simulink model "PVonGrid_patched"  (R2025a)
settings: Solver=VariableStepAuto  StartTime=0.0  StopTime=2.0  RelTol=1e-3
PreLoadFcn:
  | % Parameter basis-watt yang menghasilkan Gambar 6 pada naskah.
  | % Sama persis dengan matlab/siapkan_workspace.m. JANGAN pakai
  | % init_VIC.m: nilainya set per-unit lama dan menghasilkan respons
  | % yang sama sekali berbeda.
  | f0 = 50;  Kw = 1;  H = 4;  Ts = 1e-5;
  | num_Tdi = 1;     den_Tdi    = [0.01 1];
  | num_Tri = 1;     den_Tri    = [0.01 1];
  | num_filter = 1;  den_filter = [0.02 1];
  | Dv = 20000;      Kiv = 632;
  | clear Prated R T_filter Tdi Tri VIC_max VIC_min
undefined symbols (not defined in the file): DiscIntNeverNeededParam, Down, Ion, Lithium, Up
libraries: spsSeriesRLCBranchLib x15, mcbeeMathTransformLib x8, spsIGBTDiodeLib x5, spsCurrentMeasurementLib x4, spsVoltageMeasurementLib x4, slpidlib x3, spsThreePhaseVIMeasurementLib x3, spsMosfetLib x2, spsDiodeLib x2, spsGroundLib x2, spsUniversalBridgeLib x2, spsPower3phInstantaneousLib x2
(part 1 of 2)
settings Model: Creator=Aryo  LastModifiedBy=ASUS

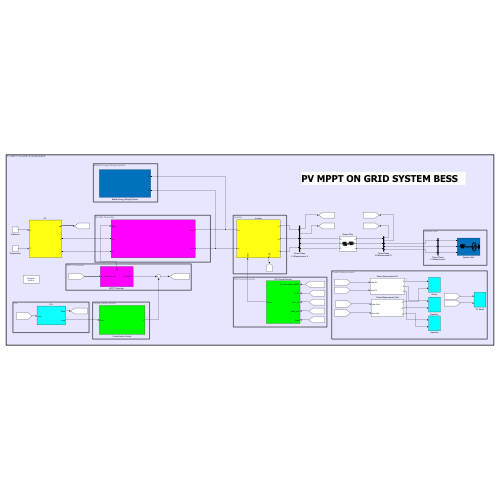
[thumbnail: Simulink's stored preview of the top-level diagram]
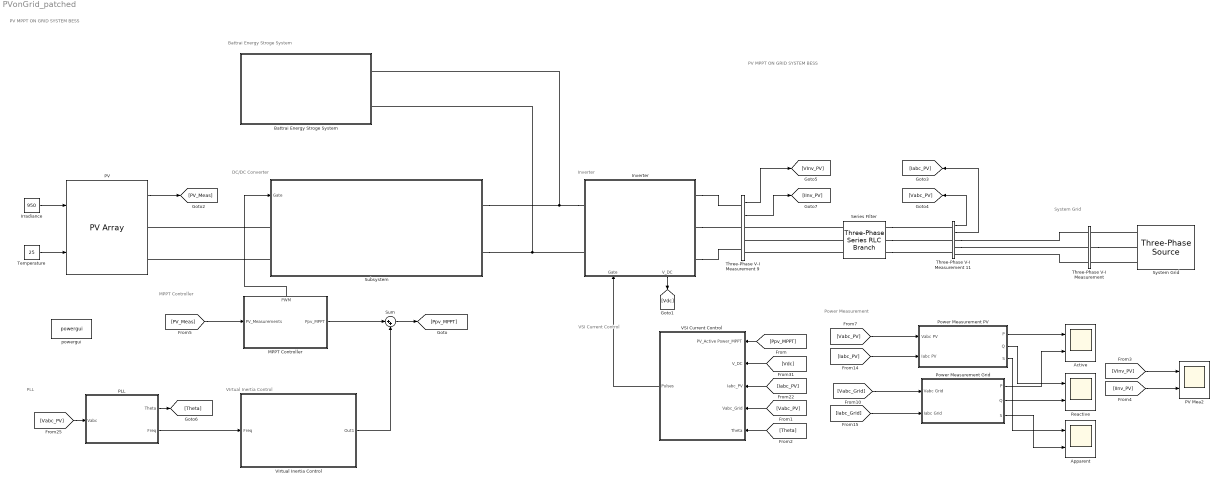
== system PVonGrid_patched ==
  note: PV MPPT ON GRID SYSTEM BESS
  note: PV MPPT ON GRID SYSTEM BESS
  note: VSI Current Control
  note: PLL
  note: Inverter
  note: Power Measurement
  note: MPPT Controller
  note: DC/DC Converter
  note: VIrtual Inertia Control
  note: Battrai Energy Stroge System
  note: System Grid
  "Active " : Scope  NumInputPorts=2
      settings: ActiveDisplayYMinimum=-60306.25275  ActiveDisplayYMaximum=6695.82422  DataLoggingVariableName=ScopeData8
  Apparent : Scope  NumInputPorts=2
      settings: ActiveDisplayYMinimum=-6789.47164  ActiveDisplayYMaximum=61149.07953  DataLoggingVariableName=ScopeData2
  Battrai Energy Stroge System : Subsystem
  Inverter : Subsystem
      settings: PortSchema="{\"entries\":[{\"content\":{\"sides\":[{\"content\":{\"connectorIds\":[\"LConn1\",\"LConn2\"]},\"type\":\"ConnectorPlacement.EquallySpacedRectSide\",\"uuid\":\"8d032cf4-7652-4960-826c-254f99f7bea5\"},{\"content\":{\"connectorIds\":[\"RConn1\",\"RConn2\",\"RConn3\"],\"side\":\"RIGHT\"},\"type\":\"ConnectorPlacement.EquallySpacedRectSide\",\"uuid\":\"6237d52f-d9ad-4fa0-b895-4b87ccfefd8d\"},{\"content\":{\"side\":\"TOP\"},\"type\":\"ConnectorPlacement.EquallySpacedRectSide\",\"uuid\":\"9697b938-6aa4-467c-bc3c-4144909828be\"},{\"content\":{\"connectorIds\":[\"In1\",\"Out1\"],\"side\":\"BOTTOM\"},\"type\":\"ConnectorPlacement.EquallySpacedRectSide\",\"uuid\":\"151792d3-0b7b-426c-bbcc-91f0e747f4d6\"}]},\"type\":\"ConnectorPlacement.EquallySpacedConnector\",\"uuid\":\"8854265a-e38a-4272-8fdc-bb8cf1e7f552\"}],\"packageUris\":[\"http://schema.mathworks.com/mf0/Connector/R2020b\"],\"version\":\"1.0\"}"
  "Irradiance " : Constant  Value=950
  MPPT Controller : Subsystem
      settings: PortSchema="{\"entries\":[{\"content\":{\"sides\":[{\"content\":{\"connectorIds\":[\"In1\"]},\"type\":\"ConnectorPlacement.EquallySpacedRectSide\",\"uuid\":\"beb56f4d-244a-4861-aa2c-056548243ef9\"},{\"content\":{\"connectorIds\":[\"Out1\"],\"side\":\"RIGHT\"},\"type\":\"ConnectorPlacement.EquallySpacedRectSide\",\"uuid\":\"efb26265-76c3-4ef7-8964-6d49d0ce5848\"},{\"content\":{\"connectorIds\":[\"Out2\"],\"side\":\"TOP\"},\"type\":\"ConnectorPlacement.EquallySpacedRectSide\",\"uuid\":\"f52004c3-ad48-43ff-bda9-03bf57742bdf\"}]},\"type\":\"ConnectorPlacement.EquallySpacedConnector\",\"uuid\":\"0b23e1d0-3529-41b8-bd5c-87ef798e8ebf\"}],\"packageUris\":[\"http://schema.mathworks.com/mf0/Connector/R2020b\"],\"version\":\"1.0\"}"
  PLL : Subsystem
  "PV " : spsPVArrayLib/PV Array  Npar=18  Nser=20  PlotType=array @ 1000 W/m2 & specified temperatures  S_vec="[ 1000  500  100 ]"  Temp_C_vec=[ 0 15 25 35 50]  ModuleName=User-defined  PlotWhenSelected=off  Pm=349.972  Ncell=96  Voc=51.7  Isc=8.65  Vm=43.1  Im=8.12  beta_Voc_pc=-0.37  alpha_Isc_pc=0.07  beta_Voc=-0.19129  alpha_Isc=0.006055  IL=8.6554  I0=4.1764e-10  nI=0.88295  Rsh=412.0293  Rs=0.25518  RobustModel=off  RobustCellTemperature=313.3991  BAL=on  Tc=1e-6  Tfilter=5e-5
  PV Mea2 : Scope  NumInputPorts=2
      settings: ActiveDisplayYMinimum=-434.46354  ActiveDisplayYMaximum=444.89351  DataLoggingVariableName=ScopeData15
  Power Measurement Grid : Subsystem
  Power Measurement PV : Subsystem
  "Reactive " : Scope  NumInputPorts=2
      settings: ActiveDisplayYMinimum=-15111.35327  ActiveDisplayYMaximum=19095.7131
  Series FIlter : spsThreePhaseSeriesRLCBranchLib/Three-Phase Series RLC Branch  LConnTagsString=A|B|C  RConnTagsString=A|B|C  BranchType=RL  Resistance=2.119394542  Inductance=10.59697271e-3  Capacitance=1e-6  Measurements=None
  Subsystem : Subsystem
  Sum : Sum  Inputs=|++
  System Grid : spsThreePhaseSourceLib/Three-Phase Source  InternalConnection=Yg  VoltagePhases=on  Voltage=380  PhaseAngle=0  Voltage_phases=[380 380 380]/sqrt(3)  PhaseAngles_phases=[0 -120 +120]  Frequency=50  NonIdealSource=on  SpecifyImpedance=off  Resistance=0  Inductance=6.56e-3  ShortCircuitLevel=100e6  BaseVoltage=380  XRratio=7  BusType=swing  Pref=1e6  Qref=0  Prefabc=[10e3, 10e3, 10e3]  Qrefabc=[0, 0, 0]  Qmin=-inf  Qmax=inf
  "Temperature " : Constant  Value=25
  "Three-Phase V-I Measurement " : spsThreePhaseVIMeasurementLib/Three-Phase V-I Measurement  VoltageMeasurement=phase-to-ground  SetLabelV=on  LabelV=Vabc_Grid  Vpu=off  VpuLL=off  CurrentMeasurement=yes  SetLabelI=on  LabelI=Iabc_Grid  Ipu=off  Pbase=100e6  Vbase=500e3  OutputType=Complex  PhasorSimulation=off  PSBequivalent=0
  Three-Phase V-I Measurement 11 : spsThreePhaseVIMeasurementLib/Three-Phase V-I Measurement  VoltageMeasurement=phase-to-ground  SetLabelV=off  LabelV=Vabc_PV  Vpu=off  VpuLL=off  CurrentMeasurement=yes  SetLabelI=off  LabelI=Iabc_PV  Ipu=off  Pbase=100e6  Vbase=500e3  OutputType=Complex  PhasorSimulation=off  PSBequivalent=0
  Three-Phase V-I Measurement 9 : spsThreePhaseVIMeasurementLib/Three-Phase V-I Measurement  VoltageMeasurement=phase-to-ground  SetLabelV=off  LabelV=VInv_PV  Vpu=off  VpuLL=off  CurrentMeasurement=yes  SetLabelI=off  LabelI=IInv_PV  Ipu=off  Pbase=100e6  Vbase=500e3  OutputType=Complex  PhasorSimulation=off  PSBequivalent=0
  VIrtual Inertia Control : Subsystem
  "VSI Current Control " : Subsystem
  powergui : sps_lib/powergui  Priority=1  SimulationMode=Discrete  SampleTime=1e-6  frequency=60  Iterations=50  frequencyindice=50  Pbase=100e6  ErrMax=1e-4  UnitsV=kV  UnitsW=MW  buscounter=0  FunctionMessages=off  echomessages=off  EnableUseOfTLC=off  CurrentSourceSwitches=off  DisableSnubberDevices=off  DisableRonSwitches=off  DisableVfSwitches=off  DisplayEquations=off  AutomaticDiscreteSolvers=off  SolverType=Tustin/Backward Euler (TBE)  Interpol=off  ExternalGateDelay=off  methode=off  Ts=100  x0status=blocks  SPID=on  SwTol=0  HookPort=off  NonlinearTolerance=1e-4  nMaxIteration=100  ContinueOnMaxIteration=off  RestoreLinks=warning  ResistiveCurrentMeasurement=off  Frange=[0:2:500]  Ylog=off  Xlog=on  ShowGrid=off  save=off  variable=ZData  structure=0  ZoomFFT=off  StartTime=0.0  cycles=1  DisplayStyle=1  fundamental=60  FreqAxis=off  MaxFrequency=1000  frequencyindicesteady=1  RmsSteady=1  display=off
  wires:
  Power Measurement Grid/1(P) -> "Active "/2
  Power Measurement Grid/3(S) -> Apparent/2
  Power Measurement Grid/2(Q) -> "Reactive "/2
  [Vabc_PV] -> Power Measurement PV/1(Vabc PV)
  [Vabc_PV] -> PLL/1(Vabc)
  [Theta] -> "VSI Current Control "/5(Theta)
  [Iabc_PV] -> "VSI Current Control "/3(Iabc_PV)
  [Iabc_PV] -> Power Measurement PV/2(Iabc PV)
  [Ppv_MPPT] -> "VSI Current Control "/1(PV_Active Power_MPPT)
  Sum/1 -> [Ppv_MPPT]
  [Vdc] -> "VSI Current Control "/2(V_DC)
  [Vabc_PV] -> "VSI Current Control "/4(Vabc_Grid)
  MPPT Controller/1(Ppv_MPPT) -> Sum/1
  VIrtual Inertia Control/1(Out1) -> Sum/2
  PLL/1(Theta) -> [Theta]
  Three-Phase V-I Measurement 11/1 -> [Vabc_PV]
  [Vabc_Grid] -> Power Measurement Grid/1(Vabc Grid)
  Inverter/1(V_DC) -> [Vdc]
  Three-Phase V-I Measurement 11/2 -> [Iabc_PV]
  Three-Phase V-I Measurement 9/2 -> [IInv_PV]
  "Irradiance "/1 -> "PV "/1
  PLL/2(Freq) -> VIrtual Inertia Control/1(Freq)
  [Iabc_Grid] -> Power Measurement Grid/2(Iabc Grid)
  "PV "/1 -> [PV_Meas]
  Three-Phase V-I Measurement 9/1 -> [VInv_PV]
  "Temperature "/1 -> "PV "/2
  Power Measurement PV/2(Q) -> "Reactive "/1
  Power Measurement PV/3(S) -> Apparent/1
  "VSI Current Control "/1(Pulses) -> Inverter/1(Gate)
  [PV_Meas] -> MPPT Controller/1(PV_Measurements)
  Power Measurement PV/1(P) -> "Active "/1
  [VInv_PV] -> PV Mea2/1
  [IInv_PV] -> PV Mea2/2
  MPPT Controller/2(PWM) -> Subsystem/1(Gate)
  connections:
  Subsystem/RConn2 -- Battrai Energy Stroge System/RConn2 -- Inverter/LConn2
  Inverter/LConn1 -- Subsystem/RConn1 -- Battrai Energy Stroge System/RConn1
  Series FIlter/RConn2 -- Three-Phase V-I Measurement 11/LConn2
  Inverter/RConn2 -- Three-Phase V-I Measurement 9/LConn2
  Inverter/RConn1 -- Three-Phase V-I Measurement 9/LConn1
  Series FIlter/RConn3 -- Three-Phase V-I Measurement 11/LConn3
  Series FIlter/LConn1 -- Three-Phase V-I Measurement 9/RConn1
  Series FIlter/LConn2 -- Three-Phase V-I Measurement 9/RConn2
  Series FIlter/LConn3 -- Three-Phase V-I Measurement 9/RConn3
  "Three-Phase V-I Measurement "/LConn3 -- Three-Phase V-I Measurement 11/RConn3
  Inverter/RConn3 -- Three-Phase V-I Measurement 9/LConn3
  Three-Phase V-I Measurement 11/RConn1 -- "Three-Phase V-I Measurement "/LConn1
  Three-Phase V-I Measurement 11/RConn2 -- "Three-Phase V-I Measurement "/LConn2
  System Grid/RConn3 -- "Three-Phase V-I Measurement "/RConn3
  Series FIlter/RConn1 -- Three-Phase V-I Measurement 11/LConn1
  "Three-Phase V-I Measurement "/RConn2 -- System Grid/RConn2
  System Grid/RConn1 -- "Three-Phase V-I Measurement "/RConn1
  Subsystem/LConn1 -- "PV "/RConn1
  Subsystem/LConn2 -- "PV "/RConn2

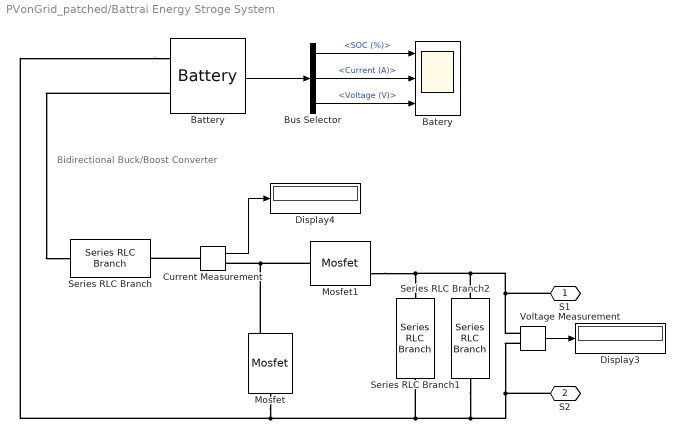
== system PVonGrid_patched/Battrai Energy Stroge System ==
  note: Bidirectional Buck/Boost Converter
  Batery : Scope  NumInputPorts=3
      settings: ActiveDisplayYMinimum=99.98642  ActiveDisplayYMaximum=100.00151  DataLoggingVariableName=ScopeData12
  Battery : spsBatteryLib/Battery  BatType=Lithium-Ion  NomV=400  NomQ=150  SOC=100  Batt_Tr=30  PresetModel=on  MaxQ=150  MinV=300  FullV=465.5949  Dis_rate=65.2174  R=0.026667  Normal_OP=135.6522  expZone="[432.1543      7.369565]"
  Bus Selector : BusSelector  OutputSignals=SOC (%),Current (A),Voltage (V)
  Current Measurement : spsCurrentMeasurementLib/Current Measurement  PhasorSimulation=off  OutputType=Complex  PSBequivalent=0
  Display3 : Display
  Display4 : Display
  Mosfet : spsMosfetLib/Mosfet  Ron=0.1  Lon=0  Rd=0.01  Vfd=0  IC=0  Rs=1e5  Cs=inf  Measurements=off
  Mosfet1 : spsMosfetLib/Mosfet  Ron=0.1  Lon=0  Rd=0.01  Vfd=0  IC=0  Rs=1e5  Cs=inf  Measurements=off
  Series RLC Branch : spsSeriesRLCBranchLib/Series RLC Branch  LConnTagsString=__new0  RConnTagsString=__new0  BranchType=L  Resistance=1  Inductance=1e-3  SetiL0=off  InitialCurrent=0  Capacitance=1e-6  Setx0=off  InitialVoltage=0  Measurements=None
  Series RLC Branch1 : spsSeriesRLCBranchLib/Series RLC Branch  LConnTagsString=__new0  RConnTagsString=__new0  BranchType=RC  Resistance=1  Inductance=1e-3  SetiL0=off  InitialCurrent=0  Capacitance=1e-6  Setx0=off  InitialVoltage=0  Measurements=None
  Series RLC Branch2 : spsSeriesRLCBranchLib/Series RLC Branch  LConnTagsString=__new0  RConnTagsString=__new0  BranchType=R  Resistance=1  Inductance=1e-3  SetiL0=off  InitialCurrent=0  Capacitance=1e-6  Setx0=off  InitialVoltage=0  Measurements=None
  Voltage Measurement : spsVoltageMeasurementLib/Voltage Measurement  PhasorSimulation=off  OutputType=Complex  PSBequivalent=0
  S1 : PMIOPort  Side=Right
  S2 : PMIOPort  Port=2  Side=Right
  wires:
  Battery/1 -> Bus Selector/1
  Voltage Measurement/1 -> Display3/1
  Current Measurement/1 -> Display4/1
  Bus Selector/3 -> Batery/3  "<Voltage (V)>"
  Bus Selector/1 -> Batery/1  "<SOC (%)>"
  Bus Selector/2 -> Batery/2  "<Current (A)>"
  connections:
  Current Measurement/RConn1 -- Mosfet/LConn1 -- Mosfet1/RConn1
  Battery/LConn2 -- Mosfet/RConn1 -- Series RLC Branch1/RConn1 -- Voltage Measurement/LConn2 -- S2/RConn1 -- Series RLC Branch2/RConn1
  S1/RConn1 -- Series RLC Branch2/LConn1 -- Series RLC Branch1/LConn1 -- Mosfet1/LConn1 -- Voltage Measurement/LConn1
  Battery/LConn1 -- Series RLC Branch/LConn1
  Current Measurement/LConn1 -- Series RLC Branch/RConn1

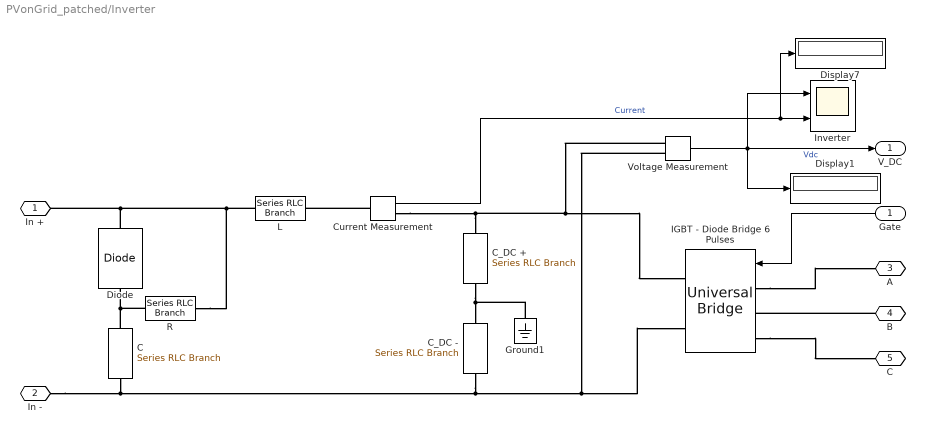
== system PVonGrid_patched/Inverter ==
  Gate : Inport
  "C " : spsSeriesRLCBranchLib/Series RLC Branch  LConnTagsString=__new0  RConnTagsString=__new0  BranchType=RC  Resistance=3e-3  Inductance=1e-3  SetiL0=off  InitialCurrent=0  Capacitance=200e-6  Setx0=off  InitialVoltage=0  Measurements=None
  C_DC + : spsSeriesRLCBranchLib/Series RLC Branch  LConnTagsString=__new0  RConnTagsString=__new0  BranchType=RC  Resistance=1e-3  Inductance=1e-3  SetiL0=off  InitialCurrent=0  Capacitance=1500e-6  Setx0=off  InitialVoltage=0  Measurements=None
  C_DC - : spsSeriesRLCBranchLib/Series RLC Branch  LConnTagsString=__new0  RConnTagsString=__new0  BranchType=RC  Resistance=1e-3  Inductance=1e-3  SetiL0=off  InitialCurrent=0  Capacitance=1500e-6  Setx0=off  InitialVoltage=0  Measurements=None
  "Current Measurement " : spsCurrentMeasurementLib/Current Measurement  PhasorSimulation=off  OutputType=Complex  PSBequivalent=0
  "Diode " : spsDiodeLib/Diode  Ron=0.001  Lon=0  Vf=1.5  IC=0  UseSnubber=0  Rs=500  Cs=250e-9  Measurements=off
  Display1 : Display
  Display7 : Display
  Ground1 : spsGroundLib/Ground  LConnTagsString=a
  IGBT - Diode Bridge 6 Pulses : spsUniversalBridgeLib/Universal Bridge  Arms=3  SnubberResistance=1e5  SnubberCapacitance=inf  Device=IGBT / Diodes  Ron=2.5e-3  Lon=0  ForwardVoltages="[  2.2  1.5  ]"  ForwardVoltage=0  GTOparameters=[ 10e-6 , 20e-6 ]  IGBTparameters=[ 1e-6 , 2e-6 ]  Measurements=None  Measurements_2=None  converterType=Rectifier
  Inverter : Scope  NumInputPorts=2
      settings: ActiveDisplayYMinimum=-86.61598  ActiveDisplayYMaximum=779.54311  DataLoggingVariableName=ScopeData11
  L : spsSeriesRLCBranchLib/Series RLC Branch  LConnTagsString=__new0  RConnTagsString=__new0  BranchType=RL  Resistance=5  Inductance=25e-3  SetiL0=off  InitialCurrent=0  Capacitance=5000e-6  Setx0=off  InitialVoltage=0  Measurements=None
  R : spsSeriesRLCBranchLib/Series RLC Branch  LConnTagsString=__new0  RConnTagsString=__new0  BranchType=R  Resistance=2  Inductance=5e-3  SetiL0=off  InitialCurrent=0  Capacitance=5000e-6  Setx0=off  InitialVoltage=0  Measurements=None
  "Voltage Measurement " : spsVoltageMeasurementLib/Voltage Measurement  PhasorSimulation=off  OutputType=Complex  PSBequivalent=0
  In + : PMIOPort  Side=Left
  In - : PMIOPort  Port=2  Side=Left
  A : PMIOPort  Port=3  Side=Right
  B : PMIOPort  Port=4  Side=Right
  C : PMIOPort  Port=5  Side=Right
  V_DC : Outport
  wires:
  Gate/1 -> IGBT - Diode Bridge 6 Pulses/1
  "Current Measurement "/1 -> Display7/1, Inverter/2  "Current"
  "Voltage Measurement "/1 -> Display1/1, Inverter/1, V_DC/1  "Vdc"
  connections:
  C_DC +/RConn1 -- Ground1/LConn1 -- C_DC -/LConn1
  L/LConn1 -- R/RConn1 -- "Diode "/LConn1 -- In +/RConn1
  C_DC +/LConn1 -- "Current Measurement "/RConn1 -- IGBT - Diode Bridge 6 Pulses/RConn1 -- "Voltage Measurement "/LConn1
  IGBT - Diode Bridge 6 Pulses/LConn1 -- A/RConn1
  IGBT - Diode Bridge 6 Pulses/LConn3 -- C/RConn1
  In -/RConn1 -- "C "/RConn1 -- C_DC -/RConn1 -- IGBT - Diode Bridge 6 Pulses/RConn2 -- "Voltage Measurement "/LConn2
  B/RConn1 -- IGBT - Diode Bridge 6 Pulses/LConn2
  "Current Measurement "/LConn1 -- L/RConn1
  "Diode "/RConn1 -- "C "/LConn1 -- R/LConn1

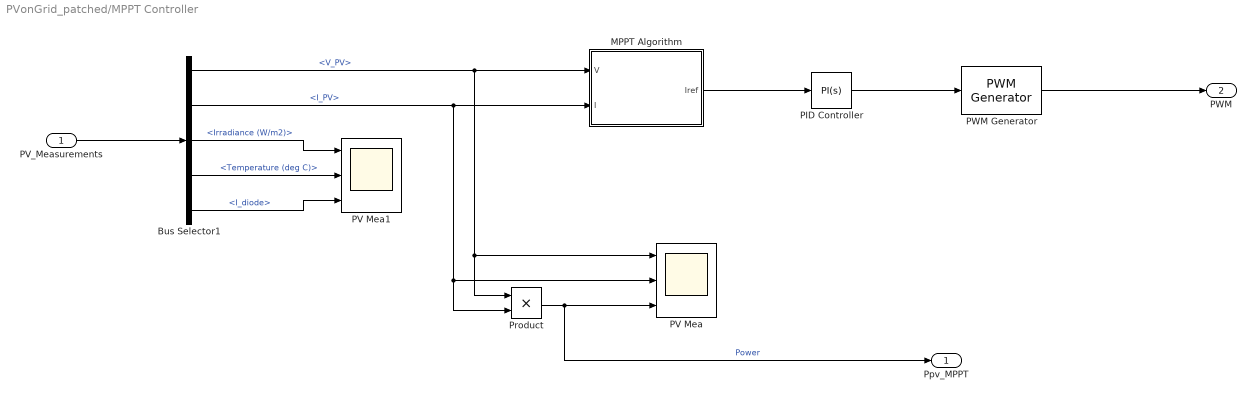
== system PVonGrid_patched/MPPT Controller ==
  PV_Measurements : Inport
  Bus Selector1 : BusSelector  OutputSignals=V_PV,I_PV,Irradiance (W/m2),Temperature (deg C),I_diode
  MPPT Algorithm : MATLAB Function  TreatAsAtomicUnit=on
  PID Controller : slpidlib/PID Controller  Controller=PI  Form=Parallel  TimeDomain=Continuous-time  UseExternalTs=off  SampleTime=-1  IntegratorMethod=Forward Euler  FilterMethod=Forward Euler  ControllerParametersSource=internal  P=0.05  I=0.05*(1/1000000)  UseKiTs=off  D=0  UseExternalDerivativeSource=off  N=100  UseFilter=on  TunerSelectOption=Transfer Function Based (PID Tuner App)  InitialConditionSource=internal  InitialConditionForIntegrator=0  InitialConditionForFilter=0  DifferentiatorICPrevScaledInput=0  ExternalReset=none  TrackingMode=off  Kt=1  LimitOutput=on  SatLimitsSource=internal  UpperSaturationLimit=1  LowerSaturationLimit=0  LinearizeAsGain=on  AntiWindupMode=none  Kb=1  LimitIntegrator=off  UpperIntegratorSaturationLimit=inf  LowerIntegratorSaturationLimit=-inf  POutMin=[]  POutMax=[]  IOutMin=[]  IOutMax=[]  DOutMin=[]  DOutMax=[]  NOutMin=[]  NOutMax=[]  SumOutMin=[]  SumOutMax=[]  SaturationOutMin=[]  SaturationOutMax=[]  PParamMin=[]  PParamMax=[]  IParamMin=[]  IParamMax=[]  DParamMin=[]  DParamMax=[]  NParamMin=[]  NParamMax=[]  KbParamMin=[]  KbParamMax=[]  KtParamMin=[]  KtParamMax=[]  KbOutMin=[]  KbOutMax=[]  KtOutMin=[]  KtOutMax=[]  IntegratorOutMin=[]  IntegratorOutMax=[]  FilterOutMin=[]  FilterOutMax=[]  SumI1OutMin=[]  SumI1OutMax=[]  SumI2OutMin=[]  SumI2OutMax=[]  SumI3OutMin=[]  SumI3OutMax=[]  SumI4OutMin=[]  SumI4OutMax=[]  SumDOutMin=[]  SumDOutMax=[]  DifferentiatorOutMin=[]  DifferentiatorOutMax=[]  FilterDiffOutCoefMin=[]  FilterDiffOutCoefMax=[]  ReciprocalOutMin=[]  ReciprocalOutMax=[]  SumDenOutMin=[]  SumDenOutMax=[]  SumNumOutMin=[]  SumNumOutMax=[]  DivideOutMin=[]  DivideOutMax=[]  UdiffTsProdOutMin=[]  UdiffTsProdOutMax=[]  NTsProdOutMin=[]  NTsProdOutMax=[]  UintegralTsProdOutMin=[]  UintegralTsProdOutMax=[]  UngainTsProdOutMin=[]  UngainTsProdOutMax=[]  ClampingZeroOutDataTypeStr=Inherit: Inherit via back propagation  ClampingZeroOutMin=[]  ClampingZeroOutMax=[]  FilterDenConstantOutDataTypeStr=Inherit: Inherit via back propagation  FilterDenConstantOutMin=[]  FilterDenConstantOutMax=[]  PCopyOutDataTypeStr=Inherit: Inherit via back propagation  PCopyOutMin=[]  PCopyOutMax=[]  NCopyOutDataTypeStr=Inherit: Inherit via back propagation  NCopyOutMin=[]  NCopyOutMax=[]  IntegratorContinuousStateAttributes=''  IntegratorStateMustResolveToSignalObject=off  IntegratorRTWStateStorageClass=Auto  FilterContinuousStateAttributes=''  FilterStateMustResolveToSignalObject=off  FilterRTWStateStorageClass=Auto  ParallelPVariant=InternalParameters  IdealPVariant=Disabled  IVariant=InternalParameters  DVariant=Disabled  IntegratorVariant=Continuous  SatVariant=Enabled  AWVariant=Passthrough  PCopyVariant=Disabled  TRVariant=Disabled  FdbkBlocksVariant=Forward  IdealPFdbkVariant=Disabled  SatFdbkVariant=Disabled  DerivativeFilterVariant=Disabled  NVariant=Disabled  NCopyVariant=Disabled_SignalSpec  FilterICVariant=Disabled  IntegratorICVariant=InternalICs  ExternalResetVariant=Disabled  TRSumVariant=Passthrough  SumFdbkVariant=Disabled  SumVariant=Sum_PI  TsampFilterVariant=InternalTs  TsampNgainVariant=Passthrough  TsampIntegralVariant=Disabled_SignalSpec  ExternalSaturationOutDataTypeStr=Inherit: Same as second input  DerivativeSourceVariant=Disabled  PreIntVariant=InternalPreInt
  PV Mea : Scope  NumInputPorts=3
      settings: ActiveDisplayYMinimum=-125.19976  ActiveDisplayYMaximum=1172.17004  DataLoggingVariableName=ScopeData13
  PV Mea1 : Scope  NumInputPorts=3
      settings: ActiveDisplayYMinimum=850  ActiveDisplayYMaximum=1050  DataLoggingVariableName=ScopeData10
  PWM Generator : eePwmGenerator/PWM Generator  CarrCount=Up-Down  Tper=1/20000  Tdelay=0  Ts=1e-6
  Product : Product
  Ppv_MPPT : Outport
  PWM : Outport  Port=2
  wires:
  PWM Generator/1 -> PWM/1
  Product/1 -> PV Mea/3, Ppv_MPPT/1  "Power"
  Bus Selector1/1 -> MPPT Algorithm/1(V), PV Mea/1, Product/1  "<V_PV>"
  Bus Selector1/2 -> PV Mea/2, Product/2, MPPT Algorithm/2(I)  "<I_PV>"
  Bus Selector1/3 -> PV Mea1/1  "<Irradiance (W/m2)>"
  Bus Selector1/5 -> PV Mea1/3  "<I_diode>"
  Bus Selector1/4 -> PV Mea1/2  "<Temperature (deg C)>"
  PV_Measurements/1 -> Bus Selector1/1
  PID Controller/1 -> PWM Generator/1
  MPPT Algorithm/1(Iref) -> PID Controller/1

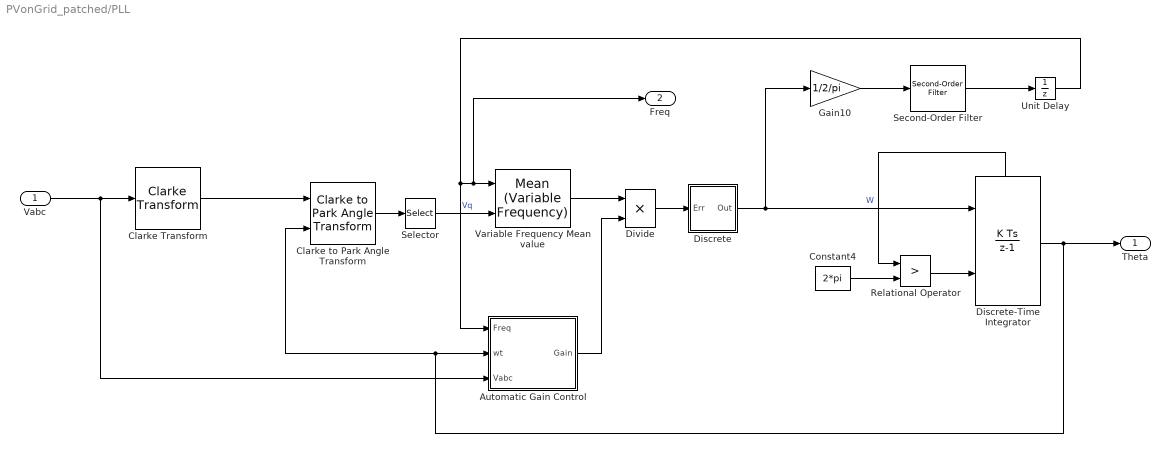
== system PVonGrid_patched/PLL ==
  Vabc : Inport
  Automatic Gain Control : Subsystem  TreatAsAtomicUnit=on
  Clarke Transform : mcbeeMathTransformLib/Clarke Transform  PowerInvariant=off  UseWithEmbedded=off  PhaseInput=Two inputs
      settings: LibrarySourceBlock=eeTransforms/Clarke Transform
  Clarke to Park Angle Transform : mcbeeMathTransformLib/Clarke to Park Angle Transform  AxisAlignment=Q-axis  UseWithEmbedded=off  PhaseInput=Two inputs  ThetaInput=Sine and Cosine electrical position  AngleInput=Per-unit  N_points=1024
      settings: LibrarySourceBlock=|
      | eeTransforms/Clarke to Park
      | Angle Transform
  Constant4 : Constant  Value=2*pi  SampleTime=1e-6
  Discrete : Subsystem  DialogController=POWERSYS.PowerSysDialog  VariantControl=PID_Discrete  mask(Discrete PID Controller){Kp=6.68450761, Ki=3.410463067, Kd=0, TcD=1e-4, Par_Limits=[inf 0], Init=2*pi*50, Ts=1e-6}
      mask prompts: Kp "Proportional gain (Kp):"; Ki "Integral gain (Ki):"; Kd "Derivative gain (Kd):"; TcD "Time constant for derivative filter (s):"; Par_Limits "Output limits: [ Upper   Lower ]"; Init "Output initial value:"; Ts "Sample time:"
      mask help: This block implements a discrete PID controller.
      mask Display: disp('PID');
  Discrete-Time Integrator : DiscreteIntegrator  ExternalReset=rising  SampleTime=1e-6  ShowStatePort=on  ICPrevOutput=DiscIntNeverNeededParam  ICPrevScaledInput=DiscIntNeverNeededParam
  Divide : Product
  Gain10 : Gain  Gain=1/2/pi  SaturateOnIntegerOverflow=on  OutDataTypeStr=Inherit: Same as input  ParamDataTypeStr=Inherit: Same as input
  Relational Operator : RelationalOperator  Operator=>  OutDataTypeStr=boolean  InputSameDT=off
  Second-Order Filter : eeGeneralControl/Second-Order Filter  FilterType=Low-pass  fn=50  Zeta=0.7  Ts=1e-6  A0=0  Ph0=0  f0=0  b0=0
  Selector : Selector  InputPortWidth=3  IndexOptions=Index vector (dialog)  Indices=2  OutputSizes=1
  Unit Delay : UnitDelay  InitialCondition=50  SampleTime=1e-6  HasFrameUpgradeWarning=on
  Variable Frequency Mean value : spsMeanVariableFrequencyLib/Mean (Variable Frequency)  Finit=50  Fmin=45  Vinit=0  Ts=1e-6
  Theta : Outport
  Freq : Outport  Port=2
  wires:
  Discrete-Time Integrator/1 -> Clarke to Park Angle Transform/2, Automatic Gain Control/2(wt), Theta/1
  Vabc/1 -> Automatic Gain Control/3(Vabc), Clarke Transform/1
  Gain10/1 -> Second-Order Filter/1
  Divide/1 -> Discrete/1(Err)
  Selector/1 -> Variable Frequency Mean value/2  "Vq"
  Clarke Transform/1 -> Clarke to Park Angle Transform/1
  Variable Frequency Mean value/1 -> Divide/1
  Clarke to Park Angle Transform/1 -> Selector/1
  Second-Order Filter/1 -> Unit Delay/1
  Discrete/1(Out) -> Discrete-Time Integrator/1, Gain10/1  "W"
  Discrete-Time Integrator/State -> Relational Operator/1
  Constant4/1 -> Relational Operator/2
  Automatic Gain Control/1(Gain) -> Divide/2
  Unit Delay/1 -> Automatic Gain Control/1(Freq), Freq/1, Variable Frequency Mean value/1
  Relational Operator/1 -> Discrete-Time Integrator/2

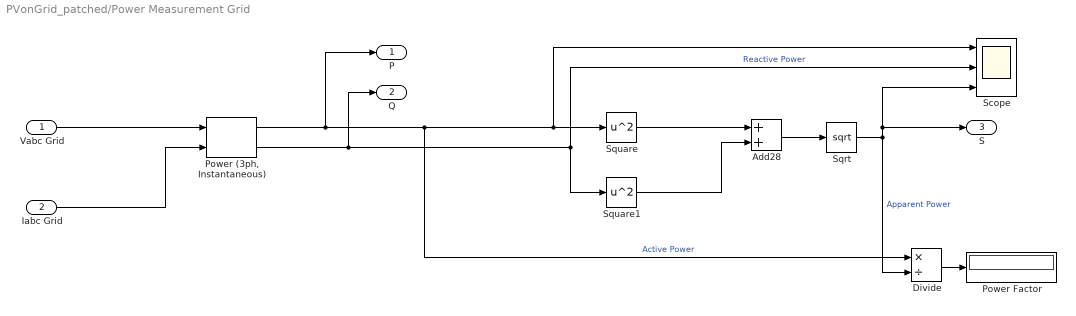
== system PVonGrid_patched/Power Measurement Grid ==
  Vabc Grid : Inport
  Iabc Grid : Inport  Port=2
  Add28 : Sum
  Divide : Product  Inputs=*/
  "Power (3ph, Instantaneous) " : spsPower3phInstantaneousLib/Power (3ph, Instantaneous)
  Power Factor : Display
  Scope : Scope  NumInputPorts=3
      settings: ActiveDisplayYMinimum=-67101.20374  ActiveDisplayYMaximum=67850.38309  DataLoggingVariableName=ScopeData5
  Sqrt : Sqrt
  Square : Math  Operator=square  SignedPower=on
  Square1 : Math  Operator=square  SignedPower=on
  P : Outport
  Q : Outport  Port=2
  S : Outport  Port=3
  wires:
  Vabc Grid/1 -> "Power (3ph, Instantaneous) "/1
  Iabc Grid/1 -> "Power (3ph, Instantaneous) "/2
  Divide/1 -> Power Factor/1
  Sqrt/1 -> Divide/2, Scope/3, S/1  "Apparent Power"
  Square1/1 -> Add28/2
  "Power (3ph, Instantaneous) "/1 -> Divide/1, Scope/1, Square/1, P/1  "Active Power"
  Square/1 -> Add28/1
  Add28/1 -> Sqrt/1
  "Power (3ph, Instantaneous) "/2 -> Q/1, Scope/2, Square1/1  "Reactive Power"

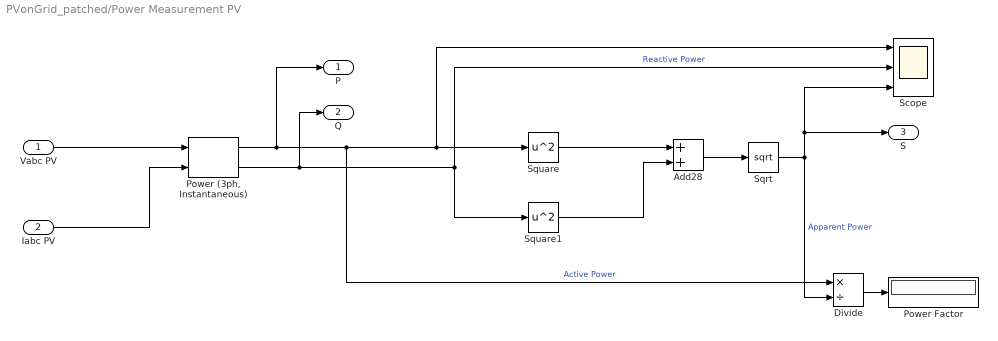
== system PVonGrid_patched/Power Measurement PV ==
  Vabc PV : Inport
  Iabc PV : Inport  Port=2
  Add28 : Sum
  Divide : Product  Inputs=*/
  "Power (3ph, Instantaneous) " : spsPower3phInstantaneousLib/Power (3ph, Instantaneous)
  Power Factor : Display
  Scope : Scope  NumInputPorts=3
      settings: ActiveDisplayYMinimum=-67101.20374  ActiveDisplayYMaximum=67850.38309  DataLoggingVariableName=ScopeData4
  Sqrt : Sqrt
  Square : Math  Operator=square  SignedPower=on
  Square1 : Math  Operator=square  SignedPower=on
  P : Outport
  Q : Outport  Port=2
  S : Outport  Port=3
  wires:
  "Power (3ph, Instantaneous) "/2 -> Scope/2, Square1/1, Q/1  "Reactive Power"
  Square1/1 -> Add28/2
  "Power (3ph, Instantaneous) "/1 -> P/1, Divide/1, Scope/1, Square/1  "Active Power"
  Iabc PV/1 -> "Power (3ph, Instantaneous) "/2
  Vabc PV/1 -> "Power (3ph, Instantaneous) "/1
  Square/1 -> Add28/1
  Sqrt/1 -> Scope/3, S/1, Divide/2  "Apparent Power"
  Add28/1 -> Sqrt/1
  Divide/1 -> Power Factor/1

== system PVonGrid_patched/Subsystem ==
  Gate : Inport
  Subsystem : Subsystem
      settings: PortSchema="{\"entries\":[{\"content\":{\"sides\":[{\"content\":{\"connectorIds\":[\"LConn1\",\"LConn2\"]},\"type\":\"ConnectorPlacement.EquallySpacedRectSide\",\"uuid\":\"91feb529-5820-4edf-8d0e-1c637fed9421\"},{\"content\":{\"connectorIds\":[\"RConn1\",\"RConn2\"],\"side\":\"RIGHT\"},\"type\":\"ConnectorPlacement.EquallySpacedRectSide\",\"uuid\":\"b4099113-c0ef-4c50-8083-88b14b98cc04\"},{\"content\":{\"side\":\"TOP\"},\"type\":\"ConnectorPlacement.EquallySpacedRectSide\",\"uuid\":\"250c6351-2de3-43d7-b6c9-3c3ed0452184\"},{\"content\":{\"connectorIds\":[\"In1\"],\"side\":\"BOTTOM\"},\"type\":\"ConnectorPlacement.EquallySpacedRectSide\",\"uuid\":\"484af620-bbf2-4328-991e-a08b15b59058\"}]},\"type\":\"ConnectorPlacement.EquallySpacedConnector\",\"uuid\":\"7041a545-1967-46d5-8643-e26f6c990daf\"}],\"packageUris\":[\"http://schema.mathworks.com/mf0/Connector/R2020b\"],\"version\":\"1.0\"}"
  Subsystem 1 : Subsystem
  Out + : PMIOPort  Side=Right
  In + : PMIOPort  Port=2  Side=Left
  Out - : PMIOPort  Port=3  Side=Right
  In - : PMIOPort  Port=4  Side=Left
  wires:
  Gate/1 -> Subsystem/1(Gate)
  [Vdc] -> Subsystem 1/1(V_DC)
  connections:
  Subsystem/RConn1 -- Subsystem 1/LConn1
  Subsystem/LConn1 -- In +/RConn1
  Subsystem/RConn2 -- Subsystem 1/LConn2
  Subsystem 1/RConn2 -- Out -/RConn1
  Subsystem 1/RConn1 -- Out +/RConn1
  Subsystem/LConn2 -- In -/RConn1

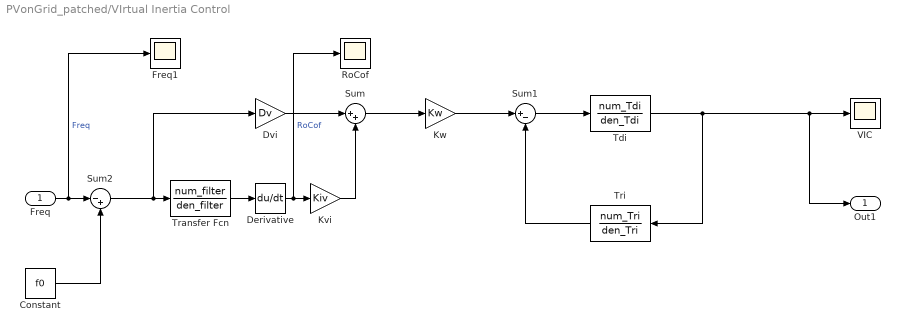
== system PVonGrid_patched/VIrtual Inertia Control ==
  Freq : Inport
  Constant : Constant  Value=f0
  Derivative : Derivative  CoefficientInTFapproximation=100
  Dvi : Gain  Gain=Dv
  Freq1 : Scope
      settings: ActiveDisplayYMinimum=-6.53762  ActiveDisplayYMaximum=58.83861  DataLoggingVariableName=ScopeData2
  Kvi : Gain  Gain=Kiv
  Kw : Gain  Gain=Kw
  RoCof : Scope
      settings: ActiveDisplayYMinimum=-172.05718  ActiveDisplayYMaximum=812.76259
  Sum : Sum  Inputs=|++
  Sum1 : Sum  Inputs=|+-
  Sum2 : Sum  Inputs=|-+
  Tdi : TransferFcn  Numerator=num_Tdi  Denominator=den_Tdi
  Transfer Fcn : TransferFcn  Numerator=num_filter  Denominator=den_filter
  Tri : TransferFcn  Numerator=num_Tri  Denominator=den_Tri
  VIC : Scope
      settings: ActiveDisplayYMinimum=-1587.17694  ActiveDisplayYMaximum=11388.49807  DataLoggingVariableName=ScopeData9
  Out1 : Outport
  wires:
  Sum/1 -> Kw/1
  Tri/1 -> Sum1/2
  Kvi/1 -> Sum/2
  Kw/1 -> Sum1/1
  Derivative/1 -> RoCof/1, Kvi/1  "RoCof"
  Sum1/1 -> Tdi/1
  Dvi/1 -> Sum/1
  Tdi/1 -> Out1/1, VIC/1, Tri/1
  Freq/1 -> Freq1/1, Sum2/1  "Freq"
  Sum2/1 -> Transfer Fcn/1, Dvi/1
  Constant/1 -> Sum2/2
  Transfer Fcn/1 -> Derivative/1

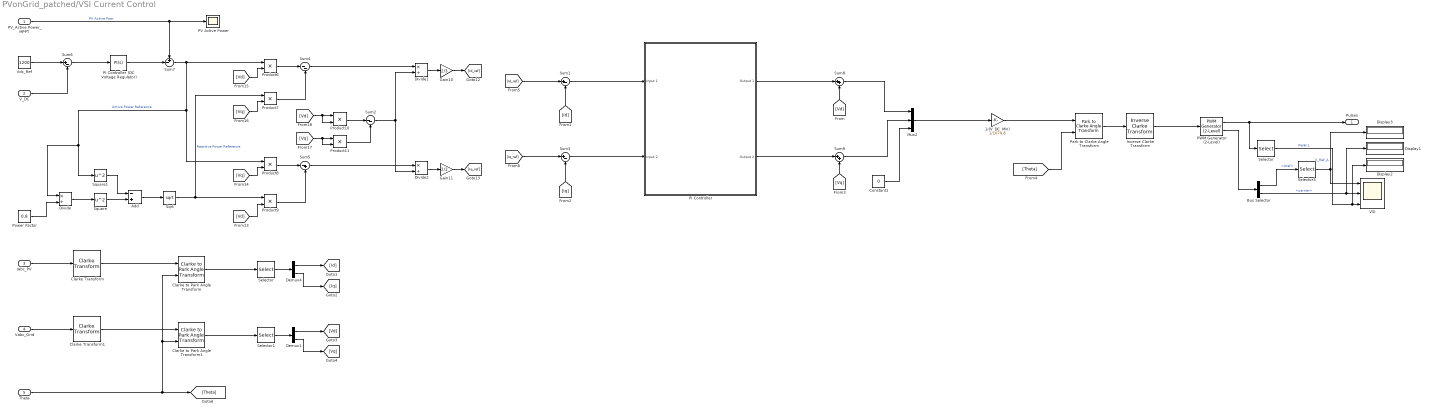
== system PVonGrid_patched/VSI Current Control  ==
  PV_Active Power_MPPT : Inport
  V_DC : Inport  Port=2
  Iabc_PV : Inport  Port=3
  Vabc_Grid : Inport  Port=4
  Theta : Inport  Port=5
  1/(V_DC_Min) : Gain  Gain=1/1074.8
  Add : Sum  Inputs=-+
  Bus Selector : BusSelector  OutputSignals=Uref,carrier
  Clarke Transform : mcbeeMathTransformLib/Clarke Transform  PowerInvariant=off  UseWithEmbedded=off  PhaseInput=Two inputs
      settings: LibrarySourceBlock=eeTransforms/Clarke Transform
  Clarke Transform1 : mcbeeMathTransformLib/Clarke Transform  PowerInvariant=off  UseWithEmbedded=off  PhaseInput=Two inputs
      settings: LibrarySourceBlock=eeTransforms/Clarke Transform
  Clarke to Park Angle Transform : mcbeeMathTransformLib/Clarke to Park Angle Transform  AxisAlignment=Q-axis  UseWithEmbedded=off  PhaseInput=Two inputs  ThetaInput=Sine and Cosine electrical position  AngleInput=Per-unit  N_points=1024
      settings: LibrarySourceBlock=|
      | eeTransforms/Clarke to Park
      | Angle Transform
  Clarke to Park Angle Transform1 : mcbeeMathTransformLib/Clarke to Park Angle Transform  AxisAlignment=Q-axis  UseWithEmbedded=off  PhaseInput=Two inputs  ThetaInput=Sine and Cosine electrical position  AngleInput=Per-unit  N_points=1024
      settings: LibrarySourceBlock=|
      | eeTransforms/Clarke to Park
      | Angle Transform
  Constant1 : Constant  Value=0
  Demux1 : Demux  Outputs=2
  Demux4 : Demux  Outputs=2
  Display1 : Display
  Display2 : Display
  Display3 : Display
  Divide : Product  Inputs=*/
  Divide1 : Product  Inputs=*/
  Divide2 : Product  Inputs=*/
  Gain10 : Gain  Gain=2/3
  Gain11 : Gain  Gain=2/3
  Inverse Clarke Transform : mcbeeMathTransformLib/Inverse Clarke Transform  PowerInvariant=off  UseWithEmbedded=off  PhaseInput=Two inputs
      settings: LibrarySourceBlock=eeTransforms/Inverse Clarke Transform
  Mux2 : Mux  Inputs=3
  PI Controller : Subsystem
  PI Controller (DC Voltage Regulator) : slpidlib/PID Controller  Controller=PI  Form=Parallel  TimeDomain=Continuous-time  UseExternalTs=off  SampleTime=1e-4  IntegratorMethod=Forward Euler  FilterMethod=Forward Euler  ControllerParametersSource=internal  P=70  I=200  UseKiTs=off  D=0  UseExternalDerivativeSource=off  N=100  UseFilter=on  TunerSelectOption=Transfer Function Based (PID Tuner App)  InitialConditionSource=internal  InitialConditionForIntegrator=0  InitialConditionForFilter=0  DifferentiatorICPrevScaledInput=0  ExternalReset=none  TrackingMode=off  Kt=1  LimitOutput=off  SatLimitsSource=internal  UpperSaturationLimit=inf  LowerSaturationLimit=-inf  LinearizeAsGain=on  AntiWindupMode=none  Kb=1  LimitIntegrator=off  UpperIntegratorSaturationLimit=inf  LowerIntegratorSaturationLimit=-inf  POutMin=[]  POutMax=[]  IOutMin=[]  IOutMax=[]  DOutMin=[]  DOutMax=[]  NOutMin=[]  NOutMax=[]  SumOutMin=[]  SumOutMax=[]  SaturationOutMin=[]  SaturationOutMax=[]  PParamMin=[]  PParamMax=[]  IParamMin=[]  IParamMax=[]  DParamMin=[]  DParamMax=[]  NParamMin=[]  NParamMax=[]  KbParamMin=[]  KbParamMax=[]  KtParamMin=[]  KtParamMax=[]  KbOutMin=[]  KbOutMax=[]  KtOutMin=[]  KtOutMax=[]  IntegratorOutMin=[]  IntegratorOutMax=[]  FilterOutMin=[]  FilterOutMax=[]  SumI1OutMin=[]  SumI1OutMax=[]  SumI2OutMin=[]  SumI2OutMax=[]  SumI3OutMin=[]  SumI3OutMax=[]  SumI4OutMin=[]  SumI4OutMax=[]  SumDOutMin=[]  SumDOutMax=[]  DifferentiatorOutMin=[]  DifferentiatorOutMax=[]  FilterDiffOutCoefMin=[]  FilterDiffOutCoefMax=[]  ReciprocalOutMin=[]  ReciprocalOutMax=[]  SumDenOutMin=[]  SumDenOutMax=[]  SumNumOutMin=[]  SumNumOutMax=[]  DivideOutMin=[]  DivideOutMax=[]  UdiffTsProdOutMin=[]  UdiffTsProdOutMax=[]  NTsProdOutMin=[]  NTsProdOutMax=[]  UintegralTsProdOutMin=[]  UintegralTsProdOutMax=[]  UngainTsProdOutMin=[]  UngainTsProdOutMax=[]  ClampingZeroOutDataTypeStr=Inherit: Inherit via back propagation  ClampingZeroOutMin=[]  ClampingZeroOutMax=[]  FilterDenConstantOutDataTypeStr=Inherit: Inherit via back propagation  FilterDenConstantOutMin=[]  FilterDenConstantOutMax=[]  PCopyOutDataTypeStr=Inherit: Inherit via back propagation  PCopyOutMin=[]  PCopyOutMax=[]  NCopyOutDataTypeStr=Inherit: Inherit via back propagation  NCopyOutMin=[]  NCopyOutMax=[]  IntegratorContinuousStateAttributes=''  IntegratorStateMustResolveToSignalObject=off  IntegratorRTWStateStorageClass=Auto  FilterContinuousStateAttributes=''  FilterStateMustResolveToSignalObject=off  FilterRTWStateStorageClass=Auto  ParallelPVariant=InternalParameters  IdealPVariant=Disabled  IVariant=InternalParameters  DVariant=Disabled  IntegratorVariant=Continuous  SatVariant=Disabled  AWVariant=Passthrough  PCopyVariant=Disabled  TRVariant=Disabled  FdbkBlocksVariant=Forward  IdealPFdbkVariant=Disabled  SatFdbkVariant=Disabled  DerivativeFilterVariant=Disabled  NVariant=Disabled  NCopyVariant=Disabled_SignalSpec  FilterICVariant=Disabled  IntegratorICVariant=InternalICs  ExternalResetVariant=Disabled  TRSumVariant=Passthrough  SumFdbkVariant=Disabled  SumVariant=Sum_PI  TsampFilterVariant=InternalTs  TsampNgainVariant=Passthrough  TsampIntegralVariant=Disabled_SignalSpec  ExternalSaturationOutDataTypeStr=Inherit: Same as second input  DerivativeSourceVariant=Disabled  PreIntVariant=InternalPreInt
  PV Active Power : Scope
      settings: ActiveDisplayYMinimum=-224286.78565  ActiveDisplayYMaximum=166336.94565  DataLoggingVariableName=ScopeData4
  "PWM Generator (2-Level) " : spsPWMGenerator2LevelLib/PWM Generator (2-Level)  ModulatorType=Three-phase bridge (6 pulses)  ModulatorMode=Unsynchronized  Fc=20000  Pc=0  nF=10000  MinMax="[ -1  1 ]"  SamplingTechnique=Natural  ModulatingSignals=off  m=0.438786204584116  Freq=50  Phase=0  Ts=1e-6  ShowCarrierOutport=on
  Park to Clarke Angle Transform : mcbeeMathTransformLib/Park to Clarke Angle Transform  AxisAlignment=Q-axis  UseWithEmbedded=off  PhaseInput=Two inputs  ThetaInput=Sine and Cosine electrical position  AngleInput=Per-unit  N_points=1024
      settings: LibrarySourceBlock=|
      | eeTransforms/Park to Clarke
      | Angle Transform
  Power Factor : Constant  Value=0.8
  Product{6..11} (6 alike) : Product
  Selector : Selector  InputPortWidth=3  IndexOptions=Index vector (dialog)  Indices=[1 2]  OutputSizes=1
  "Selector " : Selector  InputPortWidth=6  IndexOptions=Index vector (dialog)  Indices=1  OutputSizes=1
  Selector1 : Selector  InputPortWidth=3  IndexOptions=Index vector (dialog)  Indices=[1 2]  OutputSizes=1
  Selector3 : Selector  InputPortWidth=3  IndexOptions=Index vector (dialog)  Indices=1  OutputSizes=1
  Sqrt : Sqrt
  Square : Math  Operator=square
  Square1 : Math  Operator=square
  Sum1 : Sum  Inputs=|+-
  Sum2 : Sum  Inputs=|--
  Sum3 : Sum  Inputs=|+-
  Sum4 : Sum  Inputs=|--
  Sum5 : Sum  Inputs=|-+
  Sum6 : Sum  Inputs=|+-
  Sum7 : Sum  Inputs=+-|
  Sum8 : Sum  Inputs=|++
  Sum9 : Sum  Inputs=|++
  VSI : Scope  NumInputPorts=3
      settings: ActiveDisplayYMinimum=-631.87851  ActiveDisplayYMaximum=646.70919  DataLoggingVariableName=ScopeData7
  Vdc_Ref : Constant  Value=1200
  Pulses : Outport
  wires:
  Iabc_PV/1 -> Clarke Transform/1
  Clarke to Park Angle Transform/1 -> Selector/1
  Demux1/2 -> [Vq]
  Demux1/1 -> [Vd]
  Sum1/1 -> PI Controller/1(Input 1)
  Clarke to Park Angle Transform1/1 -> Selector1/1
  Theta/1 -> [Theta], Clarke to Park Angle Transform1/2, Clarke to Park Angle Transform/2
  Constant1/1 -> Mux2/3
  Vabc_Grid/1 -> Clarke Transform1/1
  Clarke Transform1/1 -> Clarke to Park Angle Transform1/1
  Clarke Transform/1 -> Clarke to Park Angle Transform/1
  Sum3/1 -> PI Controller/2(Input 2)
  Park to Clarke Angle Transform/1 -> Inverse Clarke Transform/1
  Inverse Clarke Transform/1 -> "PWM Generator (2-Level) "/1
  [Vd] -> Sum8/2
  Sum8/1 -> Mux2/1
  [Vq] -> Sum9/2
  Sum9/1 -> Mux2/2
  [Iq_ref] -> Sum3/1
  Vdc_Ref/1 -> Sum6/1
  Sum6/1 -> PI Controller (DC Voltage Regulator)/1
  V_DC/1 -> Sum6/2
  Demux4/1 -> [Id]
  Demux4/2 -> [Iq]
  [Iq] -> Sum3/2
  [Id] -> Sum1/2
  PI Controller/1(Output 1) -> Sum8/1
  PI Controller/2(Output 2) -> Sum9/1
  "PWM Generator (2-Level) "/1 -> "Selector "/1, Pulses/1
  "PWM Generator (2-Level) "/2 -> Bus Selector/1
  "Selector "/1 -> Display2/1, VSI/3  "PWM 1"
  Bus Selector/2 -> Display1/1, VSI/2  "<carrier>"
  Bus Selector/1 -> Selector3/1  "<Uref>"
  Selector3/1 -> Display3/1, VSI/1  "V_Ref_A"
  PV_Active Power_MPPT/1 -> Sum7/1, PV Active Power/1  "PV Active Poer"
  [Id_ref] -> Sum1/1
  [Theta] -> Park to Clarke Angle Transform/2
  Sqrt/1 -> Product9/1, Product7/1  "Reactive Power Reference"
  [Vd] -> Product10/1, Product10/2
  [Vd] -> Product6/2
  Sum2/1 -> Divide2/2, Divide1/2
  Product6/1 -> Sum4/1
  Product7/1 -> Sum4/2
  Sum5/1 -> Divide2/1
  [Vq] -> Product11/1, Product11/2
  Product10/1 -> Sum2/1
  Gain10/1 -> [Id_ref]
  [Vd] -> Product9/2
  [Vq] -> Product7/2
  [Vq] -> Product8/2
  Product8/1 -> Sum5/1
  Divide1/1 -> Gain10/1
  Product9/1 -> Sum5/2
  Sum4/1 -> Divide1/1
  Product11/1 -> Sum2/2
  Gain11/1 -> [Iq_ref]
  Divide2/1 -> Gain11/1
  Selector/1 -> Demux4/1
  Selector1/1 -> Demux1/1
  PI Controller (DC Voltage Regulator)/1 -> Sum7/2
  Sum7/1 -> Product6/1, Product8/1, Square1/1, Divide/1  "Active Power Reference"
  Divide/1 -> Square/1
  Power Factor/1 -> Divide/2
  Square1/1 -> Add/1
  Add/1 -> Sqrt/1
  Square/1 -> Add/2
  1/(V_DC_Min)/1 -> Park to Clarke Angle Transform/1
  Mux2/1 -> 1/(V_DC_Min)/1

== system PVonGrid_patched/PLL/Automatic Gain Control ==
  Freq : Inport
  wt : Inport  Port=2
  Vabc : Inport  Port=3
  Math Function : Math  Operator=reciprocal  SignedPower=on
  Positive-Sequence (PLL-Driven) : spsPositiveSequencePLLDrivenLib/Positive-Sequence (PLL-Driven)  Finit=50  Fmin=45  InInit=[1 0]  Ts=1e-6
  Saturation : Saturate  UpperLimit=inf  LowerLimit=0
  Terminator1 : Terminator
  Gain : Outport  InitialOutput=[1]  VectorParamsAs1DForOutWhenUnconnected=off
  wires:
  Saturation/1 -> Math Function/1
  Freq/1 -> Positive-Sequence (PLL-Driven)/1
  Vabc/1 -> Positive-Sequence (PLL-Driven)/3
  Math Function/1 -> Gain/1
  wt/1 -> Positive-Sequence (PLL-Driven)/2
  Positive-Sequence (PLL-Driven)/2 -> Terminator1/1
  Positive-Sequence (PLL-Driven)/1 -> Saturation/1

== system PVonGrid_patched/PLL/Discrete ==
  Err : Inport  SampleTime=Ts
  "Discrete Derivative " : DiscreteTransferFcn  Numerator="[ 1  -1 ]*Kd"  Denominator="[ TcD  Ts-TcD ]"  SampleTime=Ts
  Discrete-Time Integrator : DiscreteIntegrator  gainval=Ki  InitialCondition=Init  SampleTime=Ts  LimitOutput=on  UpperSaturationLimit=Par_Limits(1)  LowerSaturationLimit=Par_Limits(2)  ICPrevOutput=DiscIntNeverNeededParam  ICPrevScaledInput=DiscIntNeverNeededParam
  Kp4 : Gain  Gain=Kp  SaturateOnIntegerOverflow=on  SampleTime=Ts  OutDataTypeStr=Inherit: Same as input  ParamDataTypeStr=Inherit: Same as input
  Saturation1 : Saturate  UpperLimit=Par_Limits(1)  LowerLimit=Par_Limits(2)  SampleTime=Ts
  Sum6 : Sum  Inputs=+++  InputSameDT=on  SaturateOnIntegerOverflow=on  SampleTime=Ts  OutDataTypeStr=Inherit: Same as first input
  Out : Outport  SampleTime=Ts  InitialOutput=0  VectorParamsAs1DForOutWhenUnconnected=off
  wires:
  Saturation1/1 -> Out/1
  Err/1 -> Discrete-Time Integrator/1, Kp4/1, "Discrete Derivative "/1
  Sum6/1 -> Saturation1/1
  Kp4/1 -> Sum6/1
  Discrete-Time Integrator/1 -> Sum6/2
  "Discrete Derivative "/1 -> Sum6/3

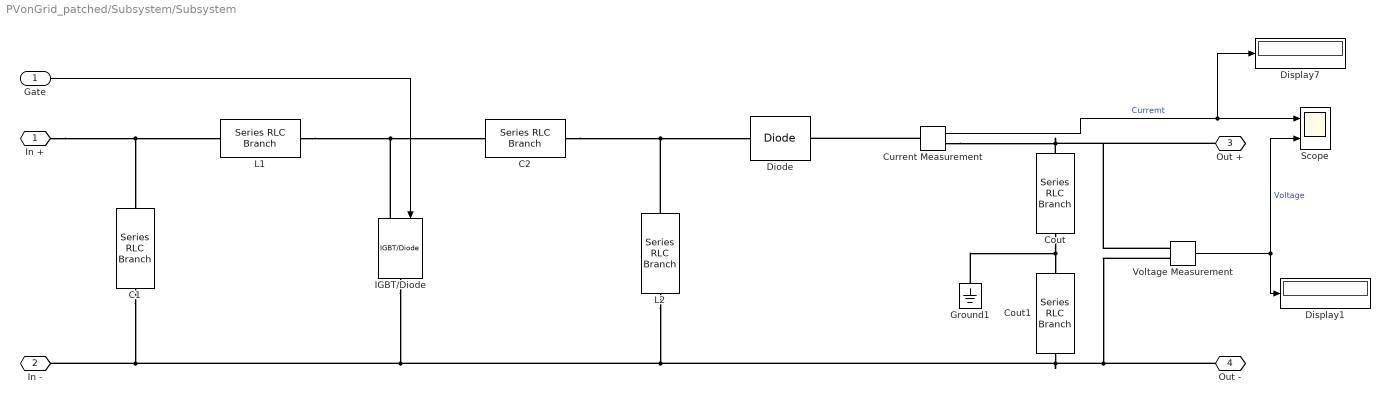
== system PVonGrid_patched/Subsystem/Subsystem ==
  Gate : Inport
  C1 : spsSeriesRLCBranchLib/Series RLC Branch  LConnTagsString=__new0  RConnTagsString=__new0  BranchType=C  Resistance=1  Inductance=1e-3  SetiL0=off  InitialCurrent=0  Capacitance=1.630974805457977e-05  Setx0=off  InitialVoltage=0  Measurements=None
  C2 : spsSeriesRLCBranchLib/Series RLC Branch  LConnTagsString=__new0  RConnTagsString=__new0  BranchType=C  Resistance=1  Inductance=1e-3  SetiL0=off  InitialCurrent=0  Capacitance=1.054425211728582e-05  Setx0=off  InitialVoltage=0  Measurements=None
  Cout : spsSeriesRLCBranchLib/Series RLC Branch  LConnTagsString=__new0  RConnTagsString=__new0  BranchType=RC  Resistance=3e-3  Inductance=16.8e-3  SetiL0=off  InitialCurrent=0  Capacitance=200e-6  Setx0=off  InitialVoltage=0  Measurements=None
  Cout1 : spsSeriesRLCBranchLib/Series RLC Branch  LConnTagsString=__new0  RConnTagsString=__new0  BranchType=RC  Resistance=3e-3  Inductance=16.8e-3  SetiL0=off  InitialCurrent=0  Capacitance=200e-6  Setx0=off  InitialVoltage=0  Measurements=None
  "Current Measurement " : spsCurrentMeasurementLib/Current Measurement  PhasorSimulation=off  OutputType=Complex  PSBequivalent=0
  "Diode " : spsDiodeLib/Diode  Ron=0.001  Lon=0  Vf=1.5  IC=0  UseSnubber=0  Rs=500  Cs=250e-9  Measurements=off
  Display1 : Display
  Display7 : Display
  Ground1 : spsGroundLib/Ground  LConnTagsString=a
  "IGBT/Diode " : spsIGBTDiodeLib/IGBT//Diode  Ron=2.5e-3  Rs=1e5  Cs=inf  Measurements=off
  L1 : spsSeriesRLCBranchLib/Series RLC Branch  LConnTagsString=__new0  RConnTagsString=__new0  BranchType=RL  Resistance=0.7  Inductance=0.003655424476162  SetiL0=off  InitialCurrent=0  Capacitance=1e-6  Setx0=off  InitialVoltage=0  Measurements=None
  L2 : spsSeriesRLCBranchLib/Series RLC Branch  LConnTagsString=__new0  RConnTagsString=__new0  BranchType=RL  Resistance=1.1  Inductance=0.005654175523838  SetiL0=off  InitialCurrent=0  Capacitance=1e-6  Setx0=off  InitialVoltage=0  Measurements=None
  Scope : Scope  NumInputPorts=2
      settings: ActiveDisplayYMinimum=-31.98832  ActiveDisplayYMaximum=250.0521  DataLoggingVariableName=ScopeData14
  "Voltage Measurement " : spsVoltageMeasurementLib/Voltage Measurement  PhasorSimulation=off  OutputType=Complex  PSBequivalent=0
  In + : PMIOPort  Side=Left
  In - : PMIOPort  Port=2  Side=Left
  Out + : PMIOPort  Port=3  Side=Right
  Out - : PMIOPort  Port=4  Side=Right
  wires:
  Gate/1 -> "IGBT/Diode "/1
  "Current Measurement "/1 -> Display7/1, Scope/1  "Curremt"
  "Voltage Measurement "/1 -> Display1/1, Scope/2  "Voltage"
  connections:
  Out -/RConn1 -- Cout1/RConn1 -- L2/RConn1 -- "IGBT/Diode "/RConn1 -- C1/RConn1 -- In -/RConn1 -- "Voltage Measurement "/LConn2
  "IGBT/Diode "/LConn1 -- L1/RConn1 -- C2/LConn1
  C2/RConn1 -- L2/LConn1 -- "Diode "/LConn1
  Cout/LConn1 -- "Voltage Measurement "/LConn1 -- Out +/RConn1 -- "Current Measurement "/RConn1
  In +/RConn1 -- L1/LConn1 -- C1/LConn1
  "Current Measurement "/LConn1 -- "Diode "/RConn1
  Cout/RConn1 -- Ground1/LConn1 -- Cout1/LConn1

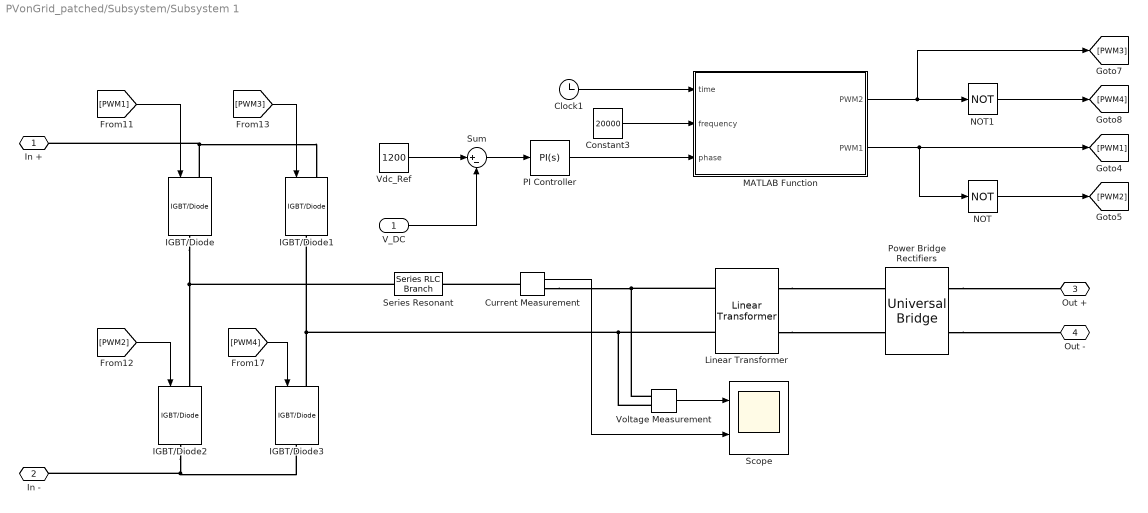
== system PVonGrid_patched/Subsystem/Subsystem 1 ==
  V_DC : Inport
  Clock1 : Clock
  Constant3 : Constant  Value=20000
  "Current Measurement " : spsCurrentMeasurementLib/Current Measurement  PhasorSimulation=off  OutputType=Complex  PSBequivalent=0
  IGBT/Diode{,1..3} (4 alike) : spsIGBTDiodeLib/IGBT//Diode  Ron=1e-3  Rs=1e5  Cs=inf  Measurements=off
  Linear Transformer : spsLinearTransformerLib/Linear Transformer  UNITS=SI  NominalPower=[ 50e3 20e3 ]  winding1=[1200 0 0]  winding2=[1200 0 0]  ThreeWindings=off  winding3=[3.15e+05 3969 1.2634]  RmLm=[14400 0.11459]  Measurements=None  DataType=on
  "MATLAB Function " : MATLAB Function  TreatAsAtomicUnit=on
  NOT : Logic  Operator=NOT  IconShape=distinctive  AllPortsSameDT=off  OutDataTypeStr=boolean
  NOT1 : Logic  Operator=NOT  IconShape=distinctive  AllPortsSameDT=off  OutDataTypeStr=boolean
  PI Controller : slpidlib/PID Controller  Controller=PI  Form=Parallel  TimeDomain=Continuous-time  UseExternalTs=off  SampleTime=-1  IntegratorMethod=Forward Euler  FilterMethod=Forward Euler  ControllerParametersSource=internal  P=100  I=1000  UseKiTs=off  D=0  UseExternalDerivativeSource=off  N=100  UseFilter=on  TunerSelectOption=Transfer Function Based (PID Tuner App)  InitialConditionSource=internal  InitialConditionForIntegrator=0  InitialConditionForFilter=0  DifferentiatorICPrevScaledInput=0  ExternalReset=none  TrackingMode=off  Kt=1  LimitOutput=on  SatLimitsSource=internal  UpperSaturationLimit=180  LowerSaturationLimit=-inf  LinearizeAsGain=on  AntiWindupMode=none  Kb=1  LimitIntegrator=off  UpperIntegratorSaturationLimit=inf  LowerIntegratorSaturationLimit=-inf  POutMin=[]  POutMax=[]  IOutMin=[]  IOutMax=[]  DOutMin=[]  DOutMax=[]  NOutMin=[]  NOutMax=[]  SumOutMin=[]  SumOutMax=[]  SaturationOutMin=[]  SaturationOutMax=[]  PParamMin=[]  PParamMax=[]  IParamMin=[]  IParamMax=[]  DParamMin=[]  DParamMax=[]  NParamMin=[]  NParamMax=[]  KbParamMin=[]  KbParamMax=[]  KtParamMin=[]  KtParamMax=[]  KbOutMin=[]  KbOutMax=[]  KtOutMin=[]  KtOutMax=[]  IntegratorOutMin=[]  IntegratorOutMax=[]  FilterOutMin=[]  FilterOutMax=[]  SumI1OutMin=[]  SumI1OutMax=[]  SumI2OutMin=[]  SumI2OutMax=[]  SumI3OutMin=[]  SumI3OutMax=[]  SumI4OutMin=[]  SumI4OutMax=[]  SumDOutMin=[]  SumDOutMax=[]  DifferentiatorOutMin=[]  DifferentiatorOutMax=[]  FilterDiffOutCoefMin=[]  FilterDiffOutCoefMax=[]  ReciprocalOutMin=[]  ReciprocalOutMax=[]  SumDenOutMin=[]  SumDenOutMax=[]  SumNumOutMin=[]  SumNumOutMax=[]  DivideOutMin=[]  DivideOutMax=[]  UdiffTsProdOutMin=[]  UdiffTsProdOutMax=[]  NTsProdOutMin=[]  NTsProdOutMax=[]  UintegralTsProdOutMin=[]  UintegralTsProdOutMax=[]  UngainTsProdOutMin=[]  UngainTsProdOutMax=[]  ClampingZeroOutDataTypeStr=Inherit: Inherit via back propagation  ClampingZeroOutMin=[]  ClampingZeroOutMax=[]  FilterDenConstantOutDataTypeStr=Inherit: Inherit via back propagation  FilterDenConstantOutMin=[]  FilterDenConstantOutMax=[]  PCopyOutDataTypeStr=Inherit: Inherit via back propagation  PCopyOutMin=[]  PCopyOutMax=[]  NCopyOutDataTypeStr=Inherit: Inherit via back propagation  NCopyOutMin=[]  NCopyOutMax=[]  IntegratorContinuousStateAttributes=''  IntegratorStateMustResolveToSignalObject=off  IntegratorRTWStateStorageClass=Auto  FilterContinuousStateAttributes=''  FilterStateMustResolveToSignalObject=off  FilterRTWStateStorageClass=Auto  ParallelPVariant=InternalParameters  IdealPVariant=Disabled  IVariant=InternalParameters  DVariant=Disabled  IntegratorVariant=Continuous  SatVariant=Enabled  AWVariant=Passthrough  PCopyVariant=Disabled  TRVariant=Disabled  FdbkBlocksVariant=Forward  IdealPFdbkVariant=Disabled  SatFdbkVariant=Disabled  DerivativeFilterVariant=Disabled  NVariant=Disabled  NCopyVariant=Disabled_SignalSpec  FilterICVariant=Disabled  IntegratorICVariant=InternalICs  ExternalResetVariant=Disabled  TRSumVariant=Passthrough  SumFdbkVariant=Disabled  SumVariant=Sum_PI  TsampFilterVariant=InternalTs  TsampNgainVariant=Passthrough  TsampIntegralVariant=Disabled_SignalSpec  ExternalSaturationOutDataTypeStr=Inherit: Same as second input  DerivativeSourceVariant=Disabled  PreIntVariant=InternalPreInt
  Power Bridge Rectifiers : spsUniversalBridgeLib/Universal Bridge  Arms=2  SnubberResistance=1e5  SnubberCapacitance=inf  Device=Diodes  Ron=1e-3  Lon=0  ForwardVoltages="[  0  0  ]"  ForwardVoltage=1.6  GTOparameters=[ 10e-6 , 20e-6 ]  IGBTparameters=[ 1e-6 , 2e-6 ]  Measurements=None  Measurements_2=None  converterType=Rectifier
  Scope : Scope  NumInputPorts=2
      settings: ActiveDisplayYMinimum=-658.88604  ActiveDisplayYMaximum=658.93522
  Series Resonant : spsSeriesRLCBranchLib/Series RLC Branch  LConnTagsString=__new0  RConnTagsString=__new0  BranchType=RLC  Resistance=0.013  Inductance=50e-6  SetiL0=off  InitialCurrent=0  Capacitance=100e-6  Setx0=off  InitialVoltage=0  Measurements=None
  Sum : Sum  Inputs=|+-
  Vdc_Ref : Constant  Value=1200
  "Voltage Measurement " : spsVoltageMeasurementLib/Voltage Measurement  PhasorSimulation=off  OutputType=Complex  PSBequivalent=0
  In + : PMIOPort  Side=Left
  In - : PMIOPort  Port=2  Side=Left
  Out + : PMIOPort  Port=3  Side=Right
  Out - : PMIOPort  Port=4  Side=Right
  wires:
  [PWM3] -> IGBT/Diode1/1
  [PWM1] -> IGBT/Diode/1
  [PWM4] -> IGBT/Diode3/1
  [PWM2] -> IGBT/Diode2/1
  V_DC/1 -> Sum/2
  PI Controller/1 -> "MATLAB Function "/3(phase)
  Vdc_Ref/1 -> Sum/1
  Constant3/1 -> "MATLAB Function "/2(frequency)
  Sum/1 -> PI Controller/1
  Clock1/1 -> "MATLAB Function "/1(time)
  "MATLAB Function "/1(PWM2) -> [PWM3], NOT1/1
  "MATLAB Function "/2(PWM1) -> [PWM1], NOT/1
  NOT/1 -> [PWM2]
  NOT1/1 -> [PWM4]
  "Voltage Measurement "/1 -> Scope/1
  "Current Measurement "/1 -> Scope/2
  connections:
  IGBT/Diode3/LConn1 -- Linear Transformer/LConn2 -- "Voltage Measurement "/LConn2 -- IGBT/Diode1/RConn1
  IGBT/Diode2/RConn1 -- In -/RConn1 -- IGBT/Diode3/RConn1
  IGBT/Diode/LConn1 -- In +/RConn1 -- IGBT/Diode1/LConn1
  Linear Transformer/RConn1 -- Power Bridge Rectifiers/LConn1
  Linear Transformer/RConn2 -- Power Bridge Rectifiers/LConn2
  Power Bridge Rectifiers/RConn1 -- Out +/RConn1
  Power Bridge Rectifiers/RConn2 -- Out -/RConn1
  IGBT/Diode/RConn1 -- Series Resonant/LConn1 -- IGBT/Diode2/LConn1
  "Current Measurement "/RConn1 -- Linear Transformer/LConn1 -- "Voltage Measurement "/LConn1
  "Current Measurement "/LConn1 -- Series Resonant/RConn1

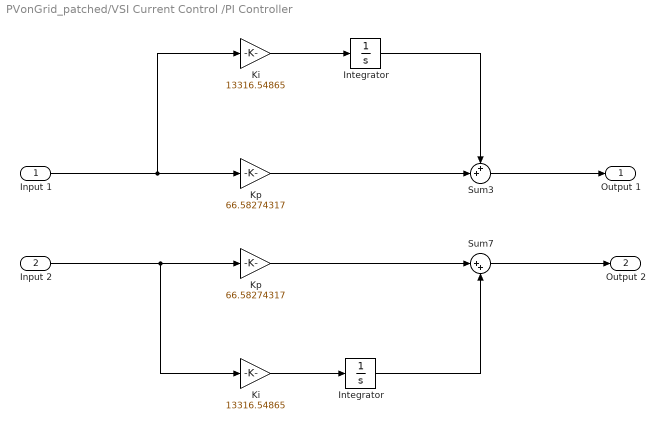
== system PVonGrid_patched/VSI Current Control /PI Controller ==
  Input 1 : Inport
  Input 2 : Inport  Port=2
  "Integrator " : Integrator
  "Integrator  " : Integrator
  Ki : Gain  Gain=13316.54865
  "Ki " : Gain  Gain=13316.54865
  Kp : Gain  Gain=66.58274317
  "Kp " : Gain  Gain=66.58274317
  Sum3 : Sum  Inputs=++|
  Sum7 : Sum  Inputs=|++
  Output 1 : Outport
  Output 2 : Outport  Port=2
  wires:
  Input 2/1 -> "Ki "/1, "Kp "/1
  "Ki "/1 -> "Integrator  "/1
  "Kp "/1 -> Sum7/1
  Kp/1 -> Sum3/2
  Sum7/1 -> Output 2/1
  Input 1/1 -> Ki/1, Kp/1
  Ki/1 -> "Integrator "/1
  Sum3/1 -> Output 1/1
  "Integrator "/1 -> Sum3/1
  "Integrator  "/1 -> Sum7/2

== matlab function PVonGrid_patched/Subsystem/Subsystem 1/MATLAB Function  ==
  data: time input; PWM2 output; frequency input; phase input; PWM1 output
function [PWM2, PWM1] = fcn(time, frequency, phase)

T_switching = 1/frequency;
PWM1 = 0;
PWM2 = 0;
x = mod(time,T_switching);

if x < T_switching/2
    PWM1 = 1;
end

t_phi = T_switching*phase/360;
y = mod(time+t_phi, T_switching);

if y < T_switching/2
    PWM2 = 1;
end
